simulink model "model"  (R2023b)
settings: Solver=VariableStepAuto  StartTime=0.0  StopTime=10.0  RelTol=1e-3
settings Model: Creator=phuryn  LastModifiedBy=phuryn

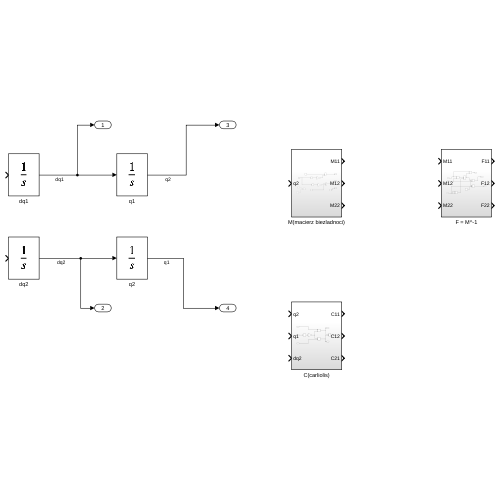
[thumbnail: Simulink's stored preview of the top-level diagram]
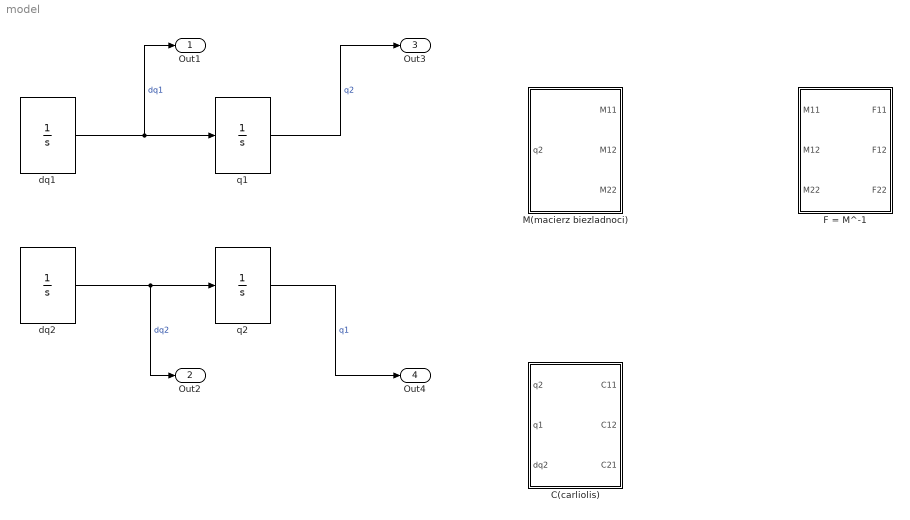
== system model ==
  C(carliolis) : Subsystem
  F = M^-1 : Subsystem
  M(macierz biezladnoci) : Subsystem
  dq1 : Integrator
  dq2 : Integrator
  q1 : Integrator
  q2 : Integrator
  Out1 : Outport
  Out2 : Outport  Port=2
  Out3 : Outport  Port=3
  Out4 : Outport  Port=4
  wires:
  dq1/1 -> Out1/1, q1/1  "dq1"
  dq2/1 -> Out2/1, q2/1  "dq2"
  q1/1 -> Out3/1  "q2"
  q2/1 -> Out4/1  "q1"

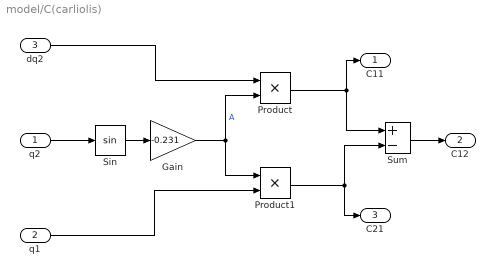
== system model/C(carliolis) ==
  q2 : Inport
  q1 : Inport  Port=2
  dq2 : Inport  Port=3
  Gain : Gain  Gain=-0.231
  Product : Product
  Product1 : Product
  Sin : Trigonometry
  Sum : Sum  Inputs=+-
  C11 : Outport
  C12 : Outport  Port=2
  C21 : Outport  Port=3
  wires:
  q2/1 -> Sin/1
  Sin/1 -> Gain/1
  Gain/1 -> Product/2, Product1/1  "A"
  Product/1 -> C11/1, Sum/1
  q1/1 -> Product1/2
  Product1/1 -> C21/1, Sum/2
  Sum/1 -> C12/1
  dq2/1 -> Product/1

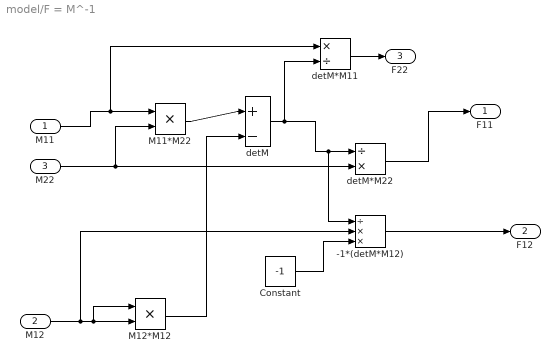
== system model/F = M^-1 ==
  M11 : Inport
  M12 : Inport  Port=2
  M22 : Inport  Port=3
  -1*(detM*M12) : Product  Inputs=/**
  Constant : Constant  Value=-1
  M11*M22 : Product
  M12*M12 : Product
  detM : Sum  Inputs=|+-
  detM*M11 : Product  Inputs=*/
  detM*M22 : Product  Inputs=/*
  F11 : Outport
  F12 : Outport  Port=2
  F22 : Outport  Port=3
  wires:
  M11/1 -> detM*M11/1, M11*M22/1
  M22/1 -> detM*M22/2, M11*M22/2
  M12/1 -> -1*(detM*M12)/2, M12*M12/2, M12*M12/1
  M11*M22/1 -> detM/1
  M12*M12/1 -> detM/2
  detM/1 -> detM*M11/2, -1*(detM*M12)/1, detM*M22/1
  detM*M22/1 -> F11/1
  -1*(detM*M12)/1 -> F12/1
  Constant/1 -> -1*(detM*M12)/3
  detM*M11/1 -> F22/1

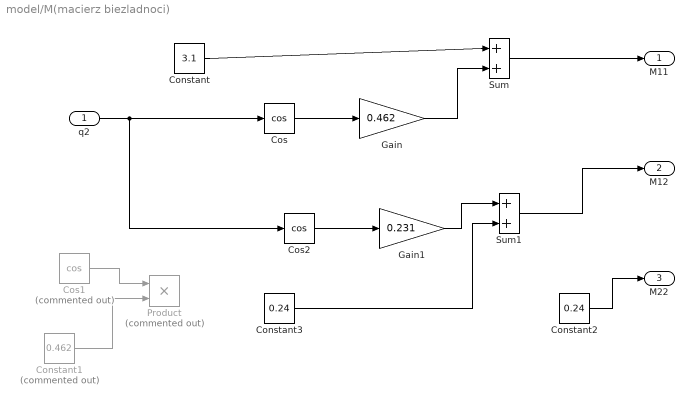
== system model/M(macierz biezladnoci) ==
  q2 : Inport
  Constant : Constant  Value=3.1
  Constant1 : Constant  Commented=on  Value=0.462
  Constant2 : Constant  Value=0.24
  Constant3 : Constant  Value=0.24
  Cos : Trigonometry  Operator=cos
  Cos1 : Trigonometry  Commented=on  Operator=cos
  Cos2 : Trigonometry  Operator=cos
  Gain : Gain  Gain=0.462
  Gain1 : Gain  Gain=0.231
  Product : Product  Commented=on
  Sum : Sum  Inputs=|++
  Sum1 : Sum  Inputs=|++
  M11 : Outport
  M12 : Outport  Port=2
  M22 : Outport  Port=3
  wires:
  Constant1/1 -> Product/2
  Cos/1 -> Gain/1
  Constant3/1 -> Sum1/2
  Gain/1 -> Sum/2
  q2/1 -> Cos2/1, Cos/1
  Cos1/1 -> Product/1
  Gain1/1 -> Sum1/1
  Cos2/1 -> Gain1/1
  Sum1/1 -> M12/1
  Constant/1 -> Sum/1
  Sum/1 -> M11/1
  Constant2/1 -> M22/1
